simulink model "animation"  (R2024b)
settings: Solver=VariableStepAuto  StartTime=0.0  StopTime=inf  RelTol=1e-3
undefined symbols (not defined in the file or in its folder): drawAircraft
settings Model: Creator=emrec  LastModifiedBy=emrec

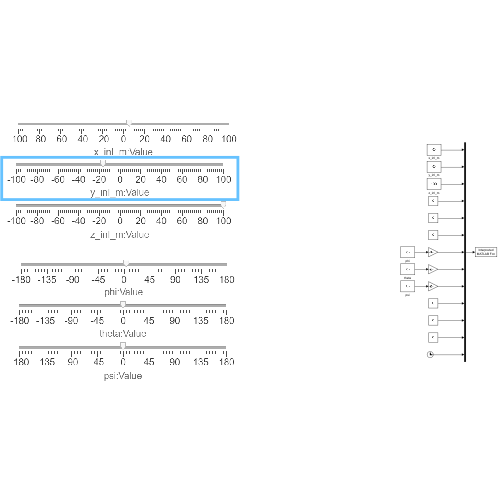
[thumbnail: Simulink's stored preview of the top-level diagram]
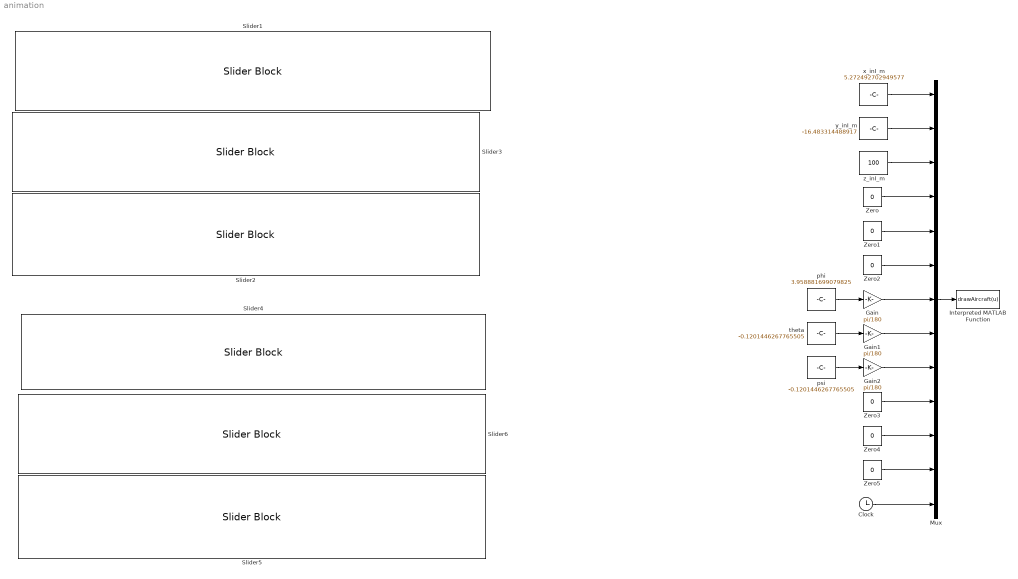
== system animation ==
  Clock : Clock
  Gain : Gain  Gain=pi/180
  Gain1 : Gain  Gain=pi/180
  Gain2 : Gain  Gain=pi/180
  Interpreted MATLAB Function : MATLABFcn  MATLABFcn=drawAircraft(u)  OutputDimensions=0
  Mux : Mux  Inputs=13
  Slider1 : SliderBlock  LabelPosition=Bottom  ScaleMin=-100  TickInterval=20
  Slider2 : SliderBlock  LabelPosition=Bottom  ScaleMin=-100  TickInterval=20
  Slider3 : SliderBlock  LabelPosition=Bottom  ScaleMin=-100  TickInterval=20
  Slider4 : SliderBlock  LabelPosition=Bottom  ScaleMin=-180  ScaleMax=180  TickInterval=45
  Slider5 : SliderBlock  LabelPosition=Bottom  ScaleMin=-180  ScaleMax=180  TickInterval=45
  Slider6 : SliderBlock  LabelPosition=Bottom  ScaleMin=-180  ScaleMax=180  TickInterval=45
  Zero{,1..5} (6 alike) : Constant  Value=0  OutDataTypeStr=Inherit: Inherit via back propagation
  phi : Constant  Value=3.958881699079825
  psi : Constant  Value=-0.1201446267765505
  theta : Constant  Value=-0.1201446267765505
  x_inI_m : Constant  Value=5.272492702949577
  y_inI_m : Constant  Value=-16.483314488917
  z_inI_m : Constant  Value=100
  wires:
  x_inI_m/1 -> Mux/1
  y_inI_m/1 -> Mux/2
  z_inI_m/1 -> Mux/3
  psi/1 -> Gain2/1
  theta/1 -> Gain1/1
  phi/1 -> Gain/1
  Zero/1 -> Mux/4
  Zero1/1 -> Mux/5
  Zero2/1 -> Mux/6
  Zero3/1 -> Mux/10
  Zero4/1 -> Mux/11
  Zero5/1 -> Mux/12
  Clock/1 -> Mux/13
  Mux/1 -> Interpreted MATLAB Function/1
  Gain/1 -> Mux/7
  Gain1/1 -> Mux/8
  Gain2/1 -> Mux/9
